simulink model "day02_forces"  (R2024a)
settings: Solver=VariableStepAuto  StartTime=0.0  StopTime=4  RelTol=1e-3
undefined symbols (not defined in the file or in its folder): g, m, T_total, v0, z0
settings Model: Creator=admin  LastModifiedBy=admin

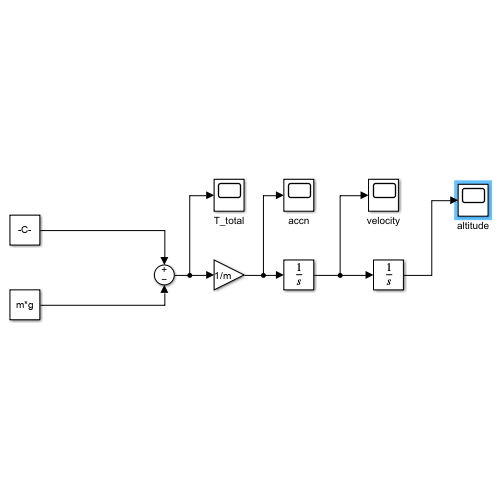
[thumbnail: Simulink's stored preview of the top-level diagram]
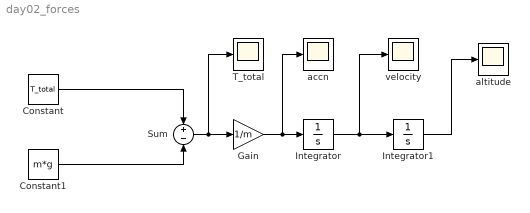
== system day02_forces ==
  Constant : Constant  Value=T_total
  Constant1 : Constant  Value=m*g
  Gain : Gain  Gain=1/m
  Integrator : Integrator  InitialCondition=v0
  Integrator1 : Integrator  InitialCondition=z0
  Sum : Sum  Inputs=+-
  T_total : Scope
  accn : Scope
  altitude : Scope
  velocity : Scope
  wires:
  Constant/1 -> Sum/1
  Constant1/1 -> Sum/2
  Sum/1 -> T_total/1, Gain/1
  Gain/1 -> accn/1, Integrator/1
  Integrator/1 -> velocity/1, Integrator1/1
  Integrator1/1 -> altitude/1
